simulink model "wturbines"  (R2024b)
settings: Solver=ode4  StartTime=0.0  StopTime=inf  FixedStep=0.01  RelTol=1e-3
values from neighbouring files (symbols this model uses):
  A_k = 2E6    (= 2000000)    [initialize_turbine_parameters.m]
  air_density = 1.225    [initialize_turbine_parameters.m]
  alpha_pitch_exp = 0    [initialize_turbine_parameters.m]
  B_k = 1E4    (= 10000)    [initialize_turbine_parameters.m]
  brake_torque = 28116.2    [initialize_turbine_parameters.m]
  C_k = 0    [initialize_turbine_parameters.m]
  Cp_mat = nan(numel(tsr_vec), numel(pitch_vec))    [initialize_turbine_parameters.m]
  Cp_opt = 0.482    [initialize_turbine_parameters.m]
  Ct_mat = nan(size(Cp_mat))    [initialize_turbine_parameters.m]
  ctrl_mode = 1    [initialize_turbine_parameters.m]
  cut_in_wind_speed = 3.0    (= 3)    [initialize_turbine_parameters.m]
  cut_out_wind_speed = 25.0    (= 25)    [initialize_turbine_parameters.m]
  D_k = 0    [initialize_turbine_parameters.m]
  dr_mode = Simulink.Parameter(1)    [initialize_turbine_parameters.m]
  gearbox_ratio = 1    [initialize_turbine_parameters.m]
  generator_eff = 0.954    [initialize_turbine_parameters.m]
  inertia = 1.9E6    (= 1900000)    [initialize_turbine_parameters.m]
  K_i_gen = 1e2    (= 100)    [initialize_turbine_parameters.m]
  K_i_pitch = 0    [initialize_turbine_parameters.m]
  K_i_pitch_gs = 0    [initialize_turbine_parameters.m]
  K_omega_sq = 1/2 * (tsr_opt)^-3 * air_density * pi * (rotor_diameter / 2)^5 * Cp_opt / gearbox_ratio^3    (= 69831977.2177)    [initialize_turbine_parameters.m]
  K_p_gen = 1e2    (= 100)    [initialize_turbine_parameters.m]
  K_p_pitch = 1    [initialize_turbine_parameters.m]
  K_p_pitch_gs = 0.1    [initialize_turbine_parameters.m]
  max_gen_torque = 1.15 * rated_gen_torque    (= 35686440.711)    [initialize_turbine_parameters.m]
  MIN_ROT_SPEED = 1e-3    (= 0.001)    [initialize_turbine_parameters.m]
  Nt = 9    [init.m]
  pitch_all = T{:, col_pitch}    [initialize_turbine_parameters.m]
  pitch_rate_deg = 5    [initialize_turbine_parameters.m]
  pitch_vec = sort(pitch_vec(:))    [initialize_turbine_parameters.m]
  rated_power = 22E6    (= 22000000)    [initialize_turbine_parameters.m]
  rated_rotor_speed = 6.77    [initialize_turbine_parameters.m]
  rated_rotor_speed_rads = rated_rotor_speed * (2 * pi) / 60    (= 0.70895274216)    [initialize_turbine_parameters.m]
  rated_wind_speed = 11.0    (= 11)    [initialize_turbine_parameters.m]
  ROT_EMG_MAX_TOL = 1.15    [initialize_turbine_parameters.m]
  ROT_SPEED_MIN_TRANS = min_rotor_speed_rads    (= 0.19)    [initialize_turbine_parameters.m]
  ROT_SPEED_SP_DIFF = 0.1    [initialize_turbine_parameters.m]
  rotor_radius = rotor_diameter / 2    (= 142)    [initialize_turbine_parameters.m]
  rotor_speed_all = [0, rated_rotor_speed]    [initialize_turbine_parameters.m]
  rotor_speed_init = rotor_speed_init * (2 * pi) / 60    (= 1.25663706144)    [initialize_turbine_parameters.m]
  rotor_speed_ref_mode = 1    [initialize_turbine_parameters.m]
  tsr_opt = 9.153    [initialize_turbine_parameters.m]
  tsr_vec = sort(tsr_vec(:))    [initialize_turbine_parameters.m]
  u_all = T{:, col_u}    [initialize_turbine_parameters.m]
  u_rotor_speed_all = [cut_in_wind_speed, rated_wind_speed]    [initialize_turbine_parameters.m]
  yawing_rate = 5    [initialize_turbine_parameters.m]
undefined symbols (not defined in the file or in its folder): op_mode, turbineDataBytes
libraries: simulink x24, simulink_extras x14, slpidlib x8, slrealtimeiplib x4, svdutilitieslib x2, slctrl_autotuning x2, etargetslib x2, dspstat3 x1
(part 2 of 3)

== system wturbines/For Each Subsystem/Turbine Dynamics + Controller1/Control logic/Power controller ==
  ws(t) : Inport
  ω(t) : Inport  Port=2
  P_set(t) : Inport  Port=3
  ω_g(t) : Inport  Port=4
  ctrl_mode : Inport  Port=5
  Demux : Demux  Outputs=2
  "Gain-scheduled H∞ control " : Subsystem
  Kω2 controller : Subsystem
  Lio downregulation : Subsystem
  Multiport Switch : MultiPortSwitch  Inputs=4  DataPortForDefault=Additional data port  SaturateOnIntegerOverflow=off  InputSameDT=off
  Mux{,1..3} (4 alike) : Mux  Inputs=2
  ROSCO : Subsystem
  T_g(t) : Outport
  β(t) : Outport  Port=2
  tag scope: ctrl_mode=global
  wires:
  Kω2 controller/1(T_g(t)) -> Mux/1
  Kω2 controller/2(β(t)) -> Mux/2
  ω(t)/1 -> Lio downregulation/1(ω(t)), "Gain-scheduled H∞ control "/1(ω_r(t))
  ws(t)/1 -> Kω2 controller/2(ws(t)), Lio downregulation/2(ws(t)), "Gain-scheduled H∞ control "/2(ws(t))
  P_set(t)/1 -> Lio downregulation/3(P_set(t))
  ctrl_mode/1 -> Multiport Switch/1, [ctrl_mode]
  Multiport Switch/1 -> Demux/1
  Demux/1 -> T_g(t)/1  "T_g(t)"
  Demux/2 -> β(t)/1  "β(t)"
  Lio downregulation/1(T_g(t)) -> Mux1/1
  Lio downregulation/2(β(t)) -> Mux1/2
  Mux/1 -> Multiport Switch/2
  Mux1/1 -> Multiport Switch/3
  ROSCO/2(β(t)) -> Mux2/2
  ROSCO/1(T_g(t)) -> Mux2/1
  "Gain-scheduled H∞ control "/1(T_g(t)) -> Mux3/1
  "Gain-scheduled H∞ control "/2(β(t)) -> Mux3/2
  Mux2/1 -> Multiport Switch/4
  Mux3/1 -> Multiport Switch/5
  ω_g(t)/1 -> Kω2 controller/1(ω(t))

== system wturbines/For Each Subsystem/Turbine Dynamics + Controller1/Turbine Dynamics/   ==
  rad : Inport
  Radians to Degrees : simulink_extras/Transformations/Radians to Degrees
  deg : Outport
  wires:
  rad/1 -> Radians to Degrees/1
  Radians to Degrees/1 -> deg/1

== system wturbines/For Each Subsystem/Turbine Dynamics + Controller1/Turbine Dynamics/      ==
  deg : Inport
  Degrees to Radians : simulink_extras/Transformations/Degrees to Radians
  rad : Outport
  wires:
  deg/1 -> Degrees to Radians/1
  Degrees to Radians/1 -> rad/1

== system wturbines/For Each Subsystem/Turbine Dynamics + Controller1/Turbine Dynamics/Collective Pitch Dynamics ==
  PtchSpt : Inport
  Rate Limiter : RateLimiter  RisingSlewLimit=pitch_rate_deg * (2 * pi / 360)  FallingSlewLimit=-pitch_rate_deg * (2 * pi / 360)  SampleTimeMode=inherited
  PitchAngle : Outport
  wires:
  PtchSpt/1 -> Rate Limiter/1
  Rate Limiter/1 -> PitchAngle/1

== system wturbines/For Each Subsystem/Turbine Dynamics + Controller1/Turbine Dynamics/Cp(λ, β) ==
  tsr : Inport
  pitch : Inport  Port=2
  Compare To Constant2 : simulink/Logic and Bit Operations/Compare To Constant  relop=<  const=min(pitch_vec)  OutDataTypeStr=boolean
  Compare To Constant3 : simulink/Logic and Bit Operations/Compare To Constant  relop=>  const=max(pitch_vec)  OutDataTypeStr=boolean
  Constant : Constant  Value=0
  "Cp(λ, β) " : Lookup_n-D  BreakpointsForDimension1=tsr_vec  BreakpointsForDimension2=pitch_vec  Table=Cp_mat  ExtrapMethod=Clip  DiagnosticForOutOfRangeInput=Error  InternalRulePriority=Speed  RndMeth=Simplest
      settings: InputPortMap=u0,u1
  OR1 : Logic  Operator=OR  IconShape=distinctive  AllPortsSameDT=off  OutDataTypeStr=boolean
  Saturation : Saturate  UpperLimit=1  LowerLimit=0
  Switch : Switch  Criteria=u2 ~= 0  SaturateOnIntegerOverflow=off  InputSameDT=off
  Cp : Outport
  wires:
  tsr/1 -> "Cp(λ, β) "/1
  pitch/1 -> "Cp(λ, β) "/2, Compare To Constant2/1, Compare To Constant3/1
  "Cp(λ, β) "/1 -> Switch/3  "Cp(t)"
  Compare To Constant2/1 -> OR1/1
  Compare To Constant3/1 -> OR1/2
  OR1/1 -> Switch/2
  Switch/1 -> Saturation/1
  Constant/1 -> Switch/1
  Saturation/1 -> Cp/1

== system wturbines/For Each Subsystem/Turbine Dynamics + Controller1/Turbine Dynamics/Orientation Dynamics ==
  OrientationSpt : Inport
  IC : InitialCondition  Value=270
  Rate Limiter : RateLimiter  RisingSlewLimit=yawing_rate  FallingSlewLimit=-yawing_rate  SampleTimeMode=inherited
  orientation : Outport
  wires:
  OrientationSpt/1 -> Rate Limiter/1  "psi_spt"
  Rate Limiter/1 -> IC/1
  IC/1 -> orientation/1

== system wturbines/For Each Subsystem/Turbine Dynamics + Controller1/Turbine Dynamics/P(t) ==
  ω(t) : Inport
  T_g(t) : Inport  Port=2
  Multiply : Gain  Gain=generator_eff
  Product : Product
  P(t) : Outport
  wires:
  ω(t)/1 -> Product/1
  T_g(t)/1 -> Product/2
  Multiply/1 -> P(t)/1
  Product/1 -> Multiply/1

== system wturbines/For Each Subsystem/Turbine Dynamics + Controller1/Turbine Dynamics/T_a(t) ==
  note: FIXME: This might have been the mistake,
      | which is fixed by this (missing) inverse
  ω(t) : Inport
  Cp(t) : Inport  Port=2
  ws(t) : Inport  Port=3
  "  " : Math  Operator=reciprocal  SignedPower=on
  Constant : Constant  Value=0.001
  Constant4 : Constant  Value=1/2
  Constant5 : Constant  Value=air_density
  Constant6 : Constant  Value=pi
  Constant7 : Constant  Value=rotor_radius
  Constant8 : Constant  Value=3
  Max : MinMax  Function=max  Inputs=2
  Power : Math  Operator=pow
  Product : Product  Inputs=7
  Saturation : Saturate  UpperLimit=inf  LowerLimit=0
  Square : Math  Operator=square
  T_a(t) : Outport
  wires:
  ω(t)/1 -> Max/1
  Product/1 -> Saturation/1  "T_a(t)"
  Square/1 -> Product/5
  Constant6/1 -> Product/6
  ws(t)/1 -> Power/1
  Constant5/1 -> Product/3
  Constant4/1 -> Product/2
  Power/1 -> Product/7
  Constant8/1 -> Power/2
  Constant7/1 -> Square/1
  Cp(t)/1 -> Product/4
  "  "/1 -> Product/1  "1/ω(t)"
  Constant/1 -> Max/2
  Max/1 -> "  "/1
  Saturation/1 -> T_a(t)/1

== system wturbines/For Each Subsystem/Turbine Dynamics + Controller1/Turbine Dynamics/λ(t) ==
  ω(t) : Inport
  ws(t) : Inport  Port=2
  Constant : Constant  Value=rotor_radius
  Divide : Product  Inputs=*/
  Product : Product
  λ(t) : Outport
  wires:
  ws(t)/1 -> Divide/2
  Product/1 -> Divide/1
  ω(t)/1 -> Product/1
  Divide/1 -> λ(t)/1  "λ(t)"
  Constant/1 -> Product/2

== system wturbines/For Each Subsystem/Turbine Dynamics + Controller/Power controller/Gain-scheduled H∞ control /  ==
  rpm : Inport
  Multiply : Gain  Gain=2 * pi
  Multiply1 : Gain  Gain=1 / 60
  rad/s : Outport
  wires:
  Multiply1/1 -> rad/s/1
  rpm/1 -> Multiply/1
  Multiply/1 -> Multiply1/1

== system wturbines/For Each Subsystem/Turbine Dynamics + Controller/Power controller/Gain-scheduled H∞ control /   ==
  rpm : Inport
  Multiply : Gain  Gain=2 * pi
  Multiply1 : Gain  Gain=1 / 60
  rad/s : Outport
  wires:
  Multiply1/1 -> rad/s/1
  rpm/1 -> Multiply/1
  Multiply/1 -> Multiply1/1

== system wturbines/For Each Subsystem/Turbine Dynamics + Controller/Power controller/Gain-scheduled H∞ control /Pitch controller ==
  e_ω,r(t) : Inport
  β(t) : Inport  Port=2
  Bus Creator : BusCreator  Inputs=2
  Gain : Gain  Gain=K_p_pitch_gs
  Gain scheduler : slctrl_autotuning/PID Gain Scheduler  ControllerType=PI  BPsInGainArray=off  GainArrayBreakpoints=[0 30]  UseExternalBreakpoints=off  GainSourceMethod=Input to block  StoreGainsPParamName=PGain  StoreGainsIParamName=IGain  StoreGainsDParamName=DGain  StoreGainsNParamName=NGain  BlockDataType=Double  PGainLookUpMeth=Interpolation-Use End Values  IGainLookUpMeth=Interpolation-Use End Values  DGainLookUpMeth=Interpolation-Use End Values  NGainLookUpMeth=Interpolation-Use End Values  DoSatur=off  BreakpointSourceLookupVariant=InternalBPs  GainSourceVariant=External  BreakpointSourceVariant=InternalBPs  PGainVariant=Enabled  IGainVariant=Enabled  DGainVariant=Disabled  NGainVariant=Disabled
      settings: LibrarySourceBlock=slctrlblks/Autotuning/PID Gain Scheduler
  Gain1 : Gain  Gain=K_i_pitch_gs
  Gains : Constant  Value=[1 3]
  PI Controller : slpidlib/PID Controller  Controller=PI  Form=Parallel  TimeDomain=Continuous-time  UseExternalTs=off  SampleTime=-1  IntegratorMethod=Forward Euler  FilterMethod=Forward Euler  ControllerParametersSource=external  P=1  I=1  UseKiTs=off  D=0  UseExternalDerivativeSource=off  N=100  UseFilter=on  TunerSelectOption=Transfer Function Based (PID Tuner App)  InitialConditionSource=internal  InitialConditionForIntegrator=0  InitialConditionForFilter=0  DifferentiatorICPrevScaledInput=0  ExternalReset=none  TrackingMode=off  Kt=1  LimitOutput=off  SatLimitsSource=internal  UpperSaturationLimit=inf  LowerSaturationLimit=-inf  LinearizeAsGain=on  AntiWindupMode=none  Kb=1  LimitIntegrator=off  UpperIntegratorSaturationLimit=inf  LowerIntegratorSaturationLimit=-inf  POutMin=[]  POutMax=[]  IOutMin=[]  IOutMax=[]  DOutMin=[]  DOutMax=[]  NOutMin=[]  NOutMax=[]  SumOutMin=[]  SumOutMax=[]  SaturationOutMin=[]  SaturationOutMax=[]  PParamMin=[]  PParamMax=[]  IParamMin=[]  IParamMax=[]  DParamMin=[]  DParamMax=[]  NParamMin=[]  NParamMax=[]  KbParamMin=[]  KbParamMax=[]  KtParamMin=[]  KtParamMax=[]  KbOutMin=[]  KbOutMax=[]  KtOutMin=[]  KtOutMax=[]  IntegratorOutMin=[]  IntegratorOutMax=[]  FilterOutMin=[]  FilterOutMax=[]  SumI1OutMin=[]  SumI1OutMax=[]  SumI2OutMin=[]  SumI2OutMax=[]  SumI3OutMin=[]  SumI3OutMax=[]  SumI4OutMin=[]  SumI4OutMax=[]  SumDOutMin=[]  SumDOutMax=[]  DifferentiatorOutMin=[]  DifferentiatorOutMax=[]  FilterDiffOutCoefMin=[]  FilterDiffOutCoefMax=[]  ReciprocalOutMin=[]  ReciprocalOutMax=[]  SumDenOutMin=[]  SumDenOutMax=[]  SumNumOutMin=[]  SumNumOutMax=[]  DivideOutMin=[]  DivideOutMax=[]  UdiffTsProdOutMin=[]  UdiffTsProdOutMax=[]  NTsProdOutMin=[]  NTsProdOutMax=[]  UintegralTsProdOutMin=[]  UintegralTsProdOutMax=[]  UngainTsProdOutMin=[]  UngainTsProdOutMax=[]  ClampingZeroOutDataTypeStr=Inherit: Inherit via back propagation  ClampingZeroOutMin=[]  ClampingZeroOutMax=[]  FilterDenConstantOutDataTypeStr=Inherit: Inherit via back propagation  FilterDenConstantOutMin=[]  FilterDenConstantOutMax=[]  PCopyOutDataTypeStr=Inherit: Inherit via back propagation  PCopyOutMin=[]  PCopyOutMax=[]  NCopyOutDataTypeStr=Inherit: Inherit via back propagation  NCopyOutMin=[]  NCopyOutMax=[]  IntegratorContinuousStateAttributes=''  IntegratorStateMustResolveToSignalObject=off  IntegratorRTWStateStorageClass=Auto  FilterContinuousStateAttributes=''  FilterStateMustResolveToSignalObject=off  FilterRTWStateStorageClass=Auto  ParallelPVariant=ExternalParameters  IdealPVariant=Disabled  IVariant=ExternalParameters  DVariant=Disabled  IntegratorVariant=Continuous  SatVariant=Disabled  AWVariant=Passthrough  PCopyVariant=Disabled  TRVariant=Disabled  FdbkBlocksVariant=Forward  IdealPFdbkVariant=Disabled  SatFdbkVariant=Disabled  DerivativeFilterVariant=Disabled  NVariant=Disabled  NCopyVariant=Disabled_SignalSpec  FilterICVariant=Disabled  IntegratorICVariant=InternalICs  ExternalResetVariant=Disabled  TRSumVariant=Passthrough  SumFdbkVariant=Disabled  SumVariant=Sum_PI  TsampFilterVariant=InternalTs  TsampNgainVariant=Passthrough  TsampIntegralVariant=Disabled_SignalSpec  ExternalSaturationOutDataTypeStr=Inherit: Same as second input  DerivativeSourceVariant=Disabled  PreIntVariant=InternalPreInt
  Signal Copy : SignalConversion  OverrideOpt=off
  rad2deg : Subsystem
  β_ref(t) : Outport
  wires:
  Signal Copy/1 -> Bus Creator/2  "I"
  β(t)/1 -> rad2deg/1(rad)
  rad2deg/1(deg) -> Gain scheduler/1  "β(t)"
  Gains/1 -> Bus Creator/1, Signal Copy/1  "P"
  Bus Creator/1 -> Gain scheduler/2
  Gain1/1 -> PI Controller/3
  Gain/1 -> PI Controller/2
  Gain scheduler/2 -> Gain1/1
  Gain scheduler/1 -> Gain/1
  PI Controller/1 -> β_ref(t)/1
  e_ω,r(t)/1 -> PI Controller/1

== system wturbines/For Each Subsystem/Turbine Dynamics + Controller/Power controller/Gain-scheduled H∞ control /Torque controller ==
  note: Temporary workaround
  e_ω,r(t) : Inport
  "H∞ controller " : StateSpace  A=A_k  B=B_k  C=C_k  D=D_k  InitialCondition=0
  PI controller : slpidlib/PID Controller  Controller=PI  Form=Parallel  TimeDomain=Continuous-time  UseExternalTs=off  SampleTime=-1  IntegratorMethod=Forward Euler  FilterMethod=Forward Euler  ControllerParametersSource=internal  P=A_k  I=B_k  UseKiTs=off  D=0  UseExternalDerivativeSource=off  N=100  UseFilter=on  TunerSelectOption=Transfer Function Based (PID Tuner App)  InitialConditionSource=internal  InitialConditionForIntegrator=0  InitialConditionForFilter=0  DifferentiatorICPrevScaledInput=0  ExternalReset=none  TrackingMode=off  Kt=1  LimitOutput=off  SatLimitsSource=internal  UpperSaturationLimit=inf  LowerSaturationLimit=-inf  LinearizeAsGain=on  AntiWindupMode=none  Kb=1  LimitIntegrator=off  UpperIntegratorSaturationLimit=inf  LowerIntegratorSaturationLimit=-inf  POutMin=[]  POutMax=[]  IOutMin=[]  IOutMax=[]  DOutMin=[]  DOutMax=[]  NOutMin=[]  NOutMax=[]  SumOutMin=[]  SumOutMax=[]  SaturationOutMin=[]  SaturationOutMax=[]  PParamMin=[]  PParamMax=[]  IParamMin=[]  IParamMax=[]  DParamMin=[]  DParamMax=[]  NParamMin=[]  NParamMax=[]  KbParamMin=[]  KbParamMax=[]  KtParamMin=[]  KtParamMax=[]  KbOutMin=[]  KbOutMax=[]  KtOutMin=[]  KtOutMax=[]  IntegratorOutMin=[]  IntegratorOutMax=[]  FilterOutMin=[]  FilterOutMax=[]  SumI1OutMin=[]  SumI1OutMax=[]  SumI2OutMin=[]  SumI2OutMax=[]  SumI3OutMin=[]  SumI3OutMax=[]  SumI4OutMin=[]  SumI4OutMax=[]  SumDOutMin=[]  SumDOutMax=[]  DifferentiatorOutMin=[]  DifferentiatorOutMax=[]  FilterDiffOutCoefMin=[]  FilterDiffOutCoefMax=[]  ReciprocalOutMin=[]  ReciprocalOutMax=[]  SumDenOutMin=[]  SumDenOutMax=[]  SumNumOutMin=[]  SumNumOutMax=[]  DivideOutMin=[]  DivideOutMax=[]  UdiffTsProdOutMin=[]  UdiffTsProdOutMax=[]  NTsProdOutMin=[]  NTsProdOutMax=[]  UintegralTsProdOutMin=[]  UintegralTsProdOutMax=[]  UngainTsProdOutMin=[]  UngainTsProdOutMax=[]  ClampingZeroOutDataTypeStr=Inherit: Inherit via back propagation  ClampingZeroOutMin=[]  ClampingZeroOutMax=[]  FilterDenConstantOutDataTypeStr=Inherit: Inherit via back propagation  FilterDenConstantOutMin=[]  FilterDenConstantOutMax=[]  PCopyOutDataTypeStr=Inherit: Inherit via back propagation  PCopyOutMin=[]  PCopyOutMax=[]  NCopyOutDataTypeStr=Inherit: Inherit via back propagation  NCopyOutMin=[]  NCopyOutMax=[]  IntegratorContinuousStateAttributes=''  IntegratorStateMustResolveToSignalObject=off  IntegratorRTWStateStorageClass=Auto  FilterContinuousStateAttributes=''  FilterStateMustResolveToSignalObject=off  FilterRTWStateStorageClass=Auto  ParallelPVariant=InternalParameters  IdealPVariant=Disabled  IVariant=InternalParameters  DVariant=Disabled  IntegratorVariant=Continuous  SatVariant=Disabled  AWVariant=Passthrough  PCopyVariant=Disabled  TRVariant=Disabled  FdbkBlocksVariant=Forward  IdealPFdbkVariant=Disabled  SatFdbkVariant=Disabled  DerivativeFilterVariant=Disabled  NVariant=Disabled  NCopyVariant=Disabled_SignalSpec  FilterICVariant=Disabled  IntegratorICVariant=InternalICs  ExternalResetVariant=Disabled  TRSumVariant=Passthrough  SumFdbkVariant=Disabled  SumVariant=Sum_PI  TsampFilterVariant=InternalTs  TsampNgainVariant=Passthrough  TsampIntegralVariant=Disabled_SignalSpec  ExternalSaturationOutDataTypeStr=Inherit: Same as second input  DerivativeSourceVariant=Disabled  PreIntVariant=InternalPreInt
  T_g(t) : Outport
  wires:
  "H∞ controller "/1 -> ?
  PI controller/1 -> T_g(t)/1
  e_ω,r(t)/1 -> PI controller/1

== system wturbines/For Each Subsystem/Turbine Dynamics + Controller/Power controller/Kω2 controller/Pitch controller ==
  ws(t) : Inport
  ω(t) : Inport  Port=2
  "  " : Subsystem
  Constant : Constant  Value=rated_rotor_speed
  Constant1 : Constant  Value=alpha_pitch_exp
  Constant2 : Constant  Value=0
  Exp : Math
  IsNaN1 : RelationalOperator  Operator=isNaN  OutDataTypeStr=boolean  RndMeth=Simplest  InputSameDT=off
  NOT : Logic  Operator=NOT  IconShape=distinctive  AllPortsSameDT=off  OutDataTypeStr=boolean
  Product : Product
  Product1 : Product
  Sum : Sum  Inputs=|+-
  Switch : Switch  Criteria=u2 ~= 0  SaturateOnIntegerOverflow=off  InputSameDT=off
  rad2deg : Subsystem
  β(ws) : Lookup_n-D  NumberOfTableDimensions=1  BreakpointsForDimension1=u_all  Table=pitch_all  InternalRulePriority=Speed  RndMeth=Simplest
  β(t) : Outport
  wires:
  Switch/1 -> β(t)/1
  NOT/1 -> Switch/2  "is_not_nan"
  Product/1 -> IsNaN1/1, Switch/1
  Constant2/1 -> Switch/3
  IsNaN1/1 -> NOT/1
  "  "/1(rad/s) -> Sum/2  "ω_rated"
  rad2deg/1(rad) -> Product/1  "β(t)"
  Constant1/1 -> Product1/2
  Product1/1 -> Exp/1
  Sum/1 -> Product1/1
  Exp/1 -> Product/2
  Constant/1 -> "  "/1(rpm)
  ω(t)/1 -> Sum/1
  ws(t)/1 -> β(ws)/1
  β(ws)/1 -> rad2deg/1(deg)

== system wturbines/For Each Subsystem/Turbine Dynamics + Controller/Power controller/Kω2 controller/Torque controller ==
  ω(t) : Inport
  Constant : Constant  Value=K_omega_sq
  Product : Product
  Square : Math  Operator=square
  T_g(t) : Outport
  wires:
  Constant/1 -> Product/2
  Product/1 -> T_g(t)/1
  Square/1 -> Product/1
  ω(t)/1 -> Square/1

== system wturbines/For Each Subsystem/Turbine Dynamics + Controller/Power controller/Lio downregulation/   ==
  rpm : Inport
  Multiply : Gain  Gain=2 * pi
  Multiply1 : Gain  Gain=1 / 60
  rad/s : Outport
  wires:
  Multiply1/1 -> rad/s/1
  rpm/1 -> Multiply/1
  Multiply/1 -> Multiply1/1

== system wturbines/For Each Subsystem/Turbine Dynamics + Controller/Power controller/Lio downregulation/Pitch controller ==
  ws(t) : Inport
  ws_dr(t) : Inport  Port=2
  e_ω(t) : Inport  Port=3
  Constant : Constant  Value=0
  Derating : Switch  Criteria=u2 > Threshold  SaturateOnIntegerOverflow=off  InputSameDT=off
  PI controller : slpidlib/PID Controller  Controller=PI  Form=Parallel  TimeDomain=Continuous-time  UseExternalTs=off  SampleTime=-1  IntegratorMethod=Forward Euler  FilterMethod=Forward Euler  ControllerParametersSource=internal  P=K_p_pitch  I=K_i_pitch  UseKiTs=off  D=0  UseExternalDerivativeSource=off  N=100  UseFilter=on  TunerSelectOption=Transfer Function Based (PID Tuner App)  InitialConditionSource=internal  InitialConditionForIntegrator=0  InitialConditionForFilter=0  DifferentiatorICPrevScaledInput=0  ExternalReset=none  TrackingMode=off  Kt=1  LimitOutput=off  SatLimitsSource=internal  UpperSaturationLimit=inf  LowerSaturationLimit=-inf  LinearizeAsGain=on  AntiWindupMode=none  Kb=1  LimitIntegrator=off  UpperIntegratorSaturationLimit=inf  LowerIntegratorSaturationLimit=-inf  POutMin=[]  POutMax=[]  IOutMin=[]  IOutMax=[]  DOutMin=[]  DOutMax=[]  NOutMin=[]  NOutMax=[]  SumOutMin=[]  SumOutMax=[]  SaturationOutMin=[]  SaturationOutMax=[]  PParamMin=[]  PParamMax=[]  IParamMin=[]  IParamMax=[]  DParamMin=[]  DParamMax=[]  NParamMin=[]  NParamMax=[]  KbParamMin=[]  KbParamMax=[]  KtParamMin=[]  KtParamMax=[]  KbOutMin=[]  KbOutMax=[]  KtOutMin=[]  KtOutMax=[]  IntegratorOutMin=[]  IntegratorOutMax=[]  FilterOutMin=[]  FilterOutMax=[]  SumI1OutMin=[]  SumI1OutMax=[]  SumI2OutMin=[]  SumI2OutMax=[]  SumI3OutMin=[]  SumI3OutMax=[]  SumI4OutMin=[]  SumI4OutMax=[]  SumDOutMin=[]  SumDOutMax=[]  DifferentiatorOutMin=[]  DifferentiatorOutMax=[]  FilterDiffOutCoefMin=[]  FilterDiffOutCoefMax=[]  ReciprocalOutMin=[]  ReciprocalOutMax=[]  SumDenOutMin=[]  SumDenOutMax=[]  SumNumOutMin=[]  SumNumOutMax=[]  DivideOutMin=[]  DivideOutMax=[]  UdiffTsProdOutMin=[]  UdiffTsProdOutMax=[]  NTsProdOutMin=[]  NTsProdOutMax=[]  UintegralTsProdOutMin=[]  UintegralTsProdOutMax=[]  UngainTsProdOutMin=[]  UngainTsProdOutMax=[]  ClampingZeroOutDataTypeStr=Inherit: Inherit via back propagation  ClampingZeroOutMin=[]  ClampingZeroOutMax=[]  FilterDenConstantOutDataTypeStr=Inherit: Inherit via back propagation  FilterDenConstantOutMin=[]  FilterDenConstantOutMax=[]  PCopyOutDataTypeStr=Inherit: Inherit via back propagation  PCopyOutMin=[]  PCopyOutMax=[]  NCopyOutDataTypeStr=Inherit: Inherit via back propagation  NCopyOutMin=[]  NCopyOutMax=[]  IntegratorContinuousStateAttributes=''  IntegratorStateMustResolveToSignalObject=off  IntegratorRTWStateStorageClass=Auto  FilterContinuousStateAttributes=''  FilterStateMustResolveToSignalObject=off  FilterRTWStateStorageClass=Auto  ParallelPVariant=InternalParameters  IdealPVariant=Disabled  IVariant=InternalParameters  DVariant=Disabled  IntegratorVariant=Continuous  SatVariant=Disabled  AWVariant=Passthrough  PCopyVariant=Disabled  TRVariant=Disabled  FdbkBlocksVariant=Forward  IdealPFdbkVariant=Disabled  SatFdbkVariant=Disabled  DerivativeFilterVariant=Disabled  NVariant=Disabled  NCopyVariant=Disabled_SignalSpec  FilterICVariant=Disabled  IntegratorICVariant=InternalICs  ExternalResetVariant=Disabled  TRSumVariant=Passthrough  SumFdbkVariant=Disabled  SumVariant=Sum_PI  TsampFilterVariant=InternalTs  TsampNgainVariant=Passthrough  TsampIntegralVariant=Disabled_SignalSpec  ExternalSaturationOutDataTypeStr=Inherit: Same as second input  DerivativeSourceVariant=Disabled  PreIntVariant=InternalPreInt
  Sum : Sum  Inputs=-+|
  β(t) : Outport
  wires:
  PI controller/1 -> Derating/3
  Constant/1 -> Derating/1
  e_ω(t)/1 -> PI controller/1
  Sum/1 -> Derating/2  "(ws_dr - ws)(t)"
  ws(t)/1 -> Sum/1
  ws_dr(t)/1 -> Sum/2
  Derating/1 -> β(t)/1

== system wturbines/For Each Subsystem/Turbine Dynamics + Controller/Power controller/Lio downregulation/Torque controller ==
  ω_set(t) : Inport
  ws(t) : Inport  Port=2
  ws_dr(t) : Inport  Port=3
  e_ω(t) : Inport  Port=4
  P_set(t) : Inport  Port=5
  Derating : Switch  Criteria=u2 > Threshold  SaturateOnIntegerOverflow=off  InputSameDT=off
  Divide : Product  Inputs=*/
  PI controller : slpidlib/PID Controller  Controller=PI  Form=Parallel  TimeDomain=Continuous-time  UseExternalTs=off  SampleTime=-1  IntegratorMethod=Forward Euler  FilterMethod=Forward Euler  ControllerParametersSource=internal  P=K_p_gen  I=K_i_gen  UseKiTs=off  D=0  UseExternalDerivativeSource=off  N=100  UseFilter=on  TunerSelectOption=Transfer Function Based (PID Tuner App)  InitialConditionSource=internal  InitialConditionForIntegrator=0  InitialConditionForFilter=0  DifferentiatorICPrevScaledInput=0  ExternalReset=none  TrackingMode=off  Kt=1  LimitOutput=off  SatLimitsSource=internal  UpperSaturationLimit=inf  LowerSaturationLimit=-inf  LinearizeAsGain=on  AntiWindupMode=none  Kb=1  LimitIntegrator=off  UpperIntegratorSaturationLimit=inf  LowerIntegratorSaturationLimit=-inf  POutMin=[]  POutMax=[]  IOutMin=[]  IOutMax=[]  DOutMin=[]  DOutMax=[]  NOutMin=[]  NOutMax=[]  SumOutMin=[]  SumOutMax=[]  SaturationOutMin=[]  SaturationOutMax=[]  PParamMin=[]  PParamMax=[]  IParamMin=[]  IParamMax=[]  DParamMin=[]  DParamMax=[]  NParamMin=[]  NParamMax=[]  KbParamMin=[]  KbParamMax=[]  KtParamMin=[]  KtParamMax=[]  KbOutMin=[]  KbOutMax=[]  KtOutMin=[]  KtOutMax=[]  IntegratorOutMin=[]  IntegratorOutMax=[]  FilterOutMin=[]  FilterOutMax=[]  SumI1OutMin=[]  SumI1OutMax=[]  SumI2OutMin=[]  SumI2OutMax=[]  SumI3OutMin=[]  SumI3OutMax=[]  SumI4OutMin=[]  SumI4OutMax=[]  SumDOutMin=[]  SumDOutMax=[]  DifferentiatorOutMin=[]  DifferentiatorOutMax=[]  FilterDiffOutCoefMin=[]  FilterDiffOutCoefMax=[]  ReciprocalOutMin=[]  ReciprocalOutMax=[]  SumDenOutMin=[]  SumDenOutMax=[]  SumNumOutMin=[]  SumNumOutMax=[]  DivideOutMin=[]  DivideOutMax=[]  UdiffTsProdOutMin=[]  UdiffTsProdOutMax=[]  NTsProdOutMin=[]  NTsProdOutMax=[]  UintegralTsProdOutMin=[]  UintegralTsProdOutMax=[]  UngainTsProdOutMin=[]  UngainTsProdOutMax=[]  ClampingZeroOutDataTypeStr=Inherit: Inherit via back propagation  ClampingZeroOutMin=[]  ClampingZeroOutMax=[]  FilterDenConstantOutDataTypeStr=Inherit: Inherit via back propagation  FilterDenConstantOutMin=[]  FilterDenConstantOutMax=[]  PCopyOutDataTypeStr=Inherit: Inherit via back propagation  PCopyOutMin=[]  PCopyOutMax=[]  NCopyOutDataTypeStr=Inherit: Inherit via back propagation  NCopyOutMin=[]  NCopyOutMax=[]  IntegratorContinuousStateAttributes=''  IntegratorStateMustResolveToSignalObject=off  IntegratorRTWStateStorageClass=Auto  FilterContinuousStateAttributes=''  FilterStateMustResolveToSignalObject=off  FilterRTWStateStorageClass=Auto  ParallelPVariant=InternalParameters  IdealPVariant=Disabled  IVariant=InternalParameters  DVariant=Disabled  IntegratorVariant=Continuous  SatVariant=Disabled  AWVariant=Passthrough  PCopyVariant=Disabled  TRVariant=Disabled  FdbkBlocksVariant=Forward  IdealPFdbkVariant=Disabled  SatFdbkVariant=Disabled  DerivativeFilterVariant=Disabled  NVariant=Disabled  NCopyVariant=Disabled_SignalSpec  FilterICVariant=Disabled  IntegratorICVariant=InternalICs  ExternalResetVariant=Disabled  TRSumVariant=Passthrough  SumFdbkVariant=Disabled  SumVariant=Sum_PI  TsampFilterVariant=InternalTs  TsampNgainVariant=Passthrough  TsampIntegralVariant=Disabled_SignalSpec  ExternalSaturationOutDataTypeStr=Inherit: Same as second input  DerivativeSourceVariant=Disabled  PreIntVariant=InternalPreInt
  Sum : Sum  Inputs=-+|
  T_g(t) : Outport
  wires:
  Divide/1 -> Derating/3
  PI controller/1 -> Derating/1
  ω_set(t)/1 -> Divide/2
  P_set(t)/1 -> Divide/1
  Derating/1 -> T_g(t)/1
  ws(t)/1 -> Sum/1
  e_ω(t)/1 -> PI controller/1
  ws_dr(t)/1 -> Sum/2
  Sum/1 -> Derating/2  "(ws_dr - ws)(t)"

== system wturbines/For Each Subsystem/Turbine Dynamics + Controller/Power controller/Lio downregulation/rads2rpm ==
  rad/s : Inport
  Multiply : Gain  Gain=1 / (2 * pi)
  Multiply1 : Gain  Gain=60
  rpm : Outport
  wires:
  Multiply1/1 -> rpm/1
  rad/s/1 -> Multiply/1
  Multiply/1 -> Multiply1/1

== system wturbines/For Each Subsystem/Turbine Dynamics + Controller/Power controller/ROSCO/Pitch controller ==
  ω_g(t) : Inport
  Δω_g(t) : Inport  Port=2
  β_min(t) : Inport  Port=3
  Constant : Constant  Value=rated_rotor_speed
  Gain : Gain  Gain=gearbox_ratio
  β(t) : Outport
  wires:
  Gain/1 -> ?  "ω_g,rated"
  Constant/1 -> Gain/1

== system wturbines/For Each Subsystem/Turbine Dynamics + Controller/Power controller/ROSCO/Torque controller ==
  ω_g(t) : Inport
  ws(t) : Inport  Port=2
  Δω_g(t) : Inport  Port=3
  β(t) : Inport  Port=4
  T_g(t) : Outport

== system wturbines/For Each Subsystem/Turbine Dynamics + Controller1/Control logic/Power controller/Gain-scheduled H∞ control  ==
  note: To prevent algebraic loop
  note: Actuator dynamics
  note: 3 | Constant-TSR
  note: 2 | Max-ω
  note: * | Shutdown
  note: 1 | Steady-state lookup
  ω_r(t) : Inport
  ws(t) : Inport  Port=2
  " " : Subsystem
  "  " : Subsystem
  Constant11 : Constant  Value=rotor_radius
  Constant12 : Constant  Value=tsr_opt
  Constant13 : Constant  Value=0
  Delay : Delay  DelayLength=1
  Divide4 : Product  Inputs=**/
  Mode : Constant  Value=rotor_speed_ref_mode
  Multiport Switch : MultiPortSwitch  DataPortForDefault=Additional data port  DiagnosticForDefault=None  SaturateOnIntegerOverflow=off  InputSameDT=off
  Pitch controller : Subsystem
  Sum : Sum  Inputs=|+-
  Torque controller : Subsystem
  ω_set : Constant  Value=rated_rotor_speed
  ω_ss(u) : Lookup_n-D  NumberOfTableDimensions=1  BreakpointsForDimension1=u_rotor_speed_all  Table=rotor_speed_all  InternalRulePriority=Speed  RndMeth=Simplest
  T_g(t) : Outport
  β(t) : Outport  Port=2
  wires:
  Torque controller/1(T_g(t)) -> T_g(t)/1
  Pitch controller/1(β_ref(t)) -> Delay/1, β(t)/1
  Delay/1 -> Pitch controller/2(β(t))
  Sum/1 -> Pitch controller/1(e_ω,r(t)), Torque controller/1(e_ω,r(t))  "e_ω,r(t)"
  Constant12/1 -> Divide4/1
  Mode/1 -> Multiport Switch/1
  Constant11/1 -> Divide4/3
  Divide4/1 -> Multiport Switch/4  "ω_r,ref(t)"
  Constant13/1 -> Multiport Switch/5
  ω_set/1 -> "  "/1(rpm)  "ω_rated"
  Multiport Switch/1 -> Sum/2  "ω_r,ref(t)"
  ω_r(t)/1 -> Sum/1
  ws(t)/1 -> ω_ss(u)/1, Divide4/2  "ws(t)"
  ω_ss(u)/1 -> " "/1(rpm)  "ω_ss(t)"
  " "/1(rad/s) -> Multiport Switch/2  "ω_ss(t)"
  "  "/1(rad/s) -> Multiport Switch/3  "ω_rated"

== system wturbines/For Each Subsystem/Turbine Dynamics + Controller1/Control logic/Power controller/Kω2 controller ==
  ω(t) : Inport
  ws(t) : Inport  Port=2
  Pitch controller : Subsystem
  Torque controller : Subsystem
  T_g(t) : Outport
  β(t) : Outport  Port=2
  wires:
  Torque controller/1(T_g(t)) -> [KomegaGen], T_g(t)/1
  Pitch controller/1(β(t)) -> β(t)/1
  ω(t)/1 -> Pitch controller/2(ω(t)), Torque controller/1(ω(t))
  ws(t)/1 -> Torque controller/2(ws), Pitch controller/1(ws(t))

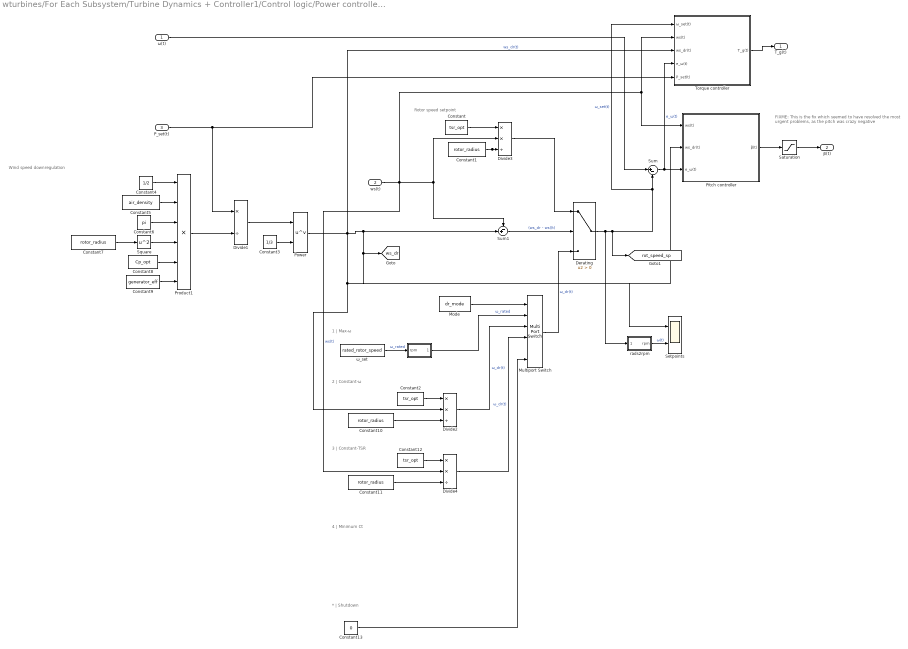
== system wturbines/For Each Subsystem/Turbine Dynamics + Controller1/Control logic/Power controller/Lio downregulation ==
  note: 1 | Max-ω
  note: Wind speed downregulation
  note: Rotor speed setpoint
  note: 2 | Constant-ω
  note: 3 | Constant-TSR
  note: 4 | Minimum Ct
  note: * | Shutdown
  note: FIXME: This is the fix which seemed to have resolved
      | the most urgent problems, as the pitch was crazy negative
  ω(t) : Inport
  ws(t) : Inport  Port=2
  P_set(t) : Inport  Port=3
  "  " : Subsystem
  Constant : Constant  Value=tsr_opt
  Constant{1,7,10..11} (4 alike) : Constant  Value=rotor_radius
  Constant12 : Constant  Value=tsr_opt
  Constant13 : Constant  Value=0
  Constant2 : Constant  Value=tsr_opt
  Constant3 : Constant  Value=1/3
  Constant4 : Constant  Value=1/2
  Constant5 : Constant  Value=air_density
  Constant6 : Constant  Value=pi
  Constant8 : Constant  Value=Cp_opt
  Constant9 : Constant  Value=generator_eff
  Derating : Switch  Criteria=u2 > Threshold  SaturateOnIntegerOverflow=off  InputSameDT=off
  Divide1 : Product  Inputs=*/
  Divide2 : Product  Inputs=**/
  Divide3 : Product  Inputs=**/
  Divide4 : Product  Inputs=**/
  Mode : Constant  Value=dr_mode
  Multiport Switch : MultiPortSwitch  Inputs=4  DataPortForDefault=Additional data port  DiagnosticForDefault=None  SaturateOnIntegerOverflow=off  InputSameDT=off
  Pitch controller : Subsystem
  Power : Math  Operator=pow
  Product1 : Product  Inputs=6
  Saturation : Saturate  UpperLimit=90 * (2 * pi / 360)  LowerLimit=-2 * (2 * pi / 360)
  Setpoints : Scope  NumInputPorts=2
  Square : Math  Operator=square
  Sum : Sum  Inputs=|+-
  Sum1 : Sum  Inputs=-+|
  Torque controller : Subsystem
  rads2rpm : Subsystem
  ω_set : Constant  Value=rated_rotor_speed
  T_g(t) : Outport
  β(t) : Outport  Port=2
  tag scope: rot_speed_sp=global, ws_dr=global
  wires:
  Torque controller/1(T_g(t)) -> T_g(t)/1
  Pitch controller/1(β(t)) -> Saturation/1
  Derating/1 -> rads2rpm/1(rad/s), Torque controller/1(ω_set(t)), Sum/2, [rot_speed_sp]  "ω_set(t)"
  Sum/1 -> Torque controller/4(e_ω(t)), Pitch controller/3(e_ω(t))  "e_ω(t)"
  Divide3/1 -> Derating/1
  Constant1/1 -> Divide3/3
  Constant/1 -> Divide3/1
  Sum1/1 -> Derating/2  "(ws_dr - ws)(t)"
  Power/1 -> Sum1/2, [ws_dr], Setpoints/1, Divide2/2, Pitch controller/2(ws_dr(t)), Torque controller/3(ws_dr(t))  "ws_dr(t)"
  ws(t)/1 -> Divide4/2, Pitch controller/1(ws(t)), Torque controller/2(ws(t)), Divide3/2, Sum1/1  "ws(t)"
  Constant3/1 -> Power/2
  P_set(t)/1 -> Torque controller/5(P_set(t)), Divide1/1
  Divide1/1 -> Power/1
  Product1/1 -> Divide1/2
  Constant4/1 -> Product1/1
  Constant5/1 -> Product1/2
  Constant6/1 -> Product1/3
  Constant7/1 -> Square/1
  Square/1 -> Product1/4
  Constant8/1 -> Product1/5
  Constant9/1 -> Product1/6
  ω(t)/1 -> Sum/1
  ω_set/1 -> "  "/1(rpm)  "ω_rated"
  Divide2/1 -> Multiport Switch/3  "ω_dr(t)"
  Constant2/1 -> Divide2/1
  Constant10/1 -> Divide2/3
  Multiport Switch/1 -> Derating/3  "ω_dr(t)"
  Mode/1 -> Multiport Switch/1
  Constant11/1 -> Divide4/3
  Constant12/1 -> Divide4/1
  Divide4/1 -> Multiport Switch/4  "ω_dr(t)"
  Constant13/1 -> Multiport Switch/6
  rads2rpm/1(rpm) -> Setpoints/2  "ω(t)"
  "  "/1(rad/s) -> Multiport Switch/2  "ω_rated"
  Saturation/1 -> β(t)/1

== system wturbines/For Each Subsystem/Turbine Dynamics + Controller1/Control logic/Power controller/ROSCO ==
  note: Setpoint smoother
  note: Pitch saturation
  ω_r(t) : Inport
  ws(t) : Inport  Port=2
  ω_g(t) : Inport  Port=3
  Pitch controller : Subsystem
  Torque controller : Subsystem
  T_g(t) : Outport
  β(t) : Outport  Port=2
  wires:
  Torque controller/1(T_g(t)) -> T_g(t)/1
  Pitch controller/1(β(t)) -> Torque controller/4(β(t)), β(t)/1
  ? -> Torque controller/3(Δω_g(t)), Pitch controller/2(Δω_g(t))  "Δω_g(t)"

== system wturbines/For Each Subsystem/Turbine Dynamics + Controller/Power controller/Gain-scheduled H∞ control /Pitch controller/rad2deg ==
  rad : Inport
  Radians to Degrees : simulink_extras/Transformations/Radians to Degrees
  deg : Outport
  wires:
  Radians to Degrees/1 -> deg/1
  rad/1 -> Radians to Degrees/1

== system wturbines/For Each Subsystem/Turbine Dynamics + Controller/Power controller/Kω2 controller/Pitch controller/   ==
  rpm : Inport
  Multiply : Gain  Gain=2 * pi
  Multiply1 : Gain  Gain=1 / 60
  rad/s : Outport
  wires:
  Multiply1/1 -> rad/s/1
  rpm/1 -> Multiply/1
  Multiply/1 -> Multiply1/1

== system wturbines/For Each Subsystem/Turbine Dynamics + Controller/Power controller/Kω2 controller/Pitch controller/rad2deg ==
  deg : Inport
  Degrees to Radians : simulink_extras/Transformations/Degrees to Radians
  rad : Outport
  wires:
  Degrees to Radians/1 -> rad/1
  deg/1 -> Degrees to Radians/1

== system wturbines/For Each Subsystem/Turbine Dynamics + Controller1/Control logic/Power controller/Gain-scheduled H∞ control /  ==
  rpm : Inport
  Multiply : Gain  Gain=2 * pi
  Multiply1 : Gain  Gain=1 / 60
  rad/s : Outport
  wires:
  Multiply/1 -> Multiply1/1
  rpm/1 -> Multiply/1
  Multiply1/1 -> rad/s/1

== system wturbines/For Each Subsystem/Turbine Dynamics + Controller1/Control logic/Power controller/Gain-scheduled H∞ control /   ==
  rpm : Inport
  Multiply : Gain  Gain=2 * pi
  Multiply1 : Gain  Gain=1 / 60
  rad/s : Outport
  wires:
  Multiply/1 -> Multiply1/1
  rpm/1 -> Multiply/1
  Multiply1/1 -> rad/s/1

== system wturbines/For Each Subsystem/Turbine Dynamics + Controller1/Control logic/Power controller/Gain-scheduled H∞ control /Pitch controller ==
  e_ω,r(t) : Inport
  β(t) : Inport  Port=2
  Bus Creator : BusCreator  Inputs=2
  Gain : Gain  Gain=K_p_pitch_gs
  Gain scheduler : slctrl_autotuning/PID Gain Scheduler  ControllerType=PI  BPsInGainArray=off  GainArrayBreakpoints=[0 30]  UseExternalBreakpoints=off  GainSourceMethod=Input to block  StoreGainsPParamName=PGain  StoreGainsIParamName=IGain  StoreGainsDParamName=DGain  StoreGainsNParamName=NGain  BlockDataType=Double  PGainLookUpMeth=Interpolation-Use End Values  IGainLookUpMeth=Interpolation-Use End Values  DGainLookUpMeth=Interpolation-Use End Values  NGainLookUpMeth=Interpolation-Use End Values  DoSatur=off  BreakpointSourceLookupVariant=InternalBPs  GainSourceVariant=External  BreakpointSourceVariant=InternalBPs  PGainVariant=Enabled  IGainVariant=Enabled  DGainVariant=Disabled  NGainVariant=Disabled
      settings: LibrarySourceBlock=slctrlblks/Autotuning/PID Gain Scheduler
  Gain1 : Gain  Gain=K_i_pitch_gs
  Gains : Constant  Value=[1 3]
  PI Controller : slpidlib/PID Controller  Controller=PI  Form=Parallel  TimeDomain=Continuous-time  UseExternalTs=off  SampleTime=-1  IntegratorMethod=Forward Euler  FilterMethod=Forward Euler  ControllerParametersSource=external  P=1  I=1  UseKiTs=off  D=0  UseExternalDerivativeSource=off  N=100  UseFilter=on  TunerSelectOption=Transfer Function Based (PID Tuner App)  InitialConditionSource=internal  InitialConditionForIntegrator=0  InitialConditionForFilter=0  DifferentiatorICPrevScaledInput=0  ExternalReset=none  TrackingMode=off  Kt=1  LimitOutput=off  SatLimitsSource=internal  UpperSaturationLimit=inf  LowerSaturationLimit=-inf  LinearizeAsGain=on  AntiWindupMode=none  Kb=1  LimitIntegrator=off  UpperIntegratorSaturationLimit=inf  LowerIntegratorSaturationLimit=-inf  POutMin=[]  POutMax=[]  IOutMin=[]  IOutMax=[]  DOutMin=[]  DOutMax=[]  NOutMin=[]  NOutMax=[]  SumOutMin=[]  SumOutMax=[]  SaturationOutMin=[]  SaturationOutMax=[]  PParamMin=[]  PParamMax=[]  IParamMin=[]  IParamMax=[]  DParamMin=[]  DParamMax=[]  NParamMin=[]  NParamMax=[]  KbParamMin=[]  KbParamMax=[]  KtParamMin=[]  KtParamMax=[]  KbOutMin=[]  KbOutMax=[]  KtOutMin=[]  KtOutMax=[]  IntegratorOutMin=[]  IntegratorOutMax=[]  FilterOutMin=[]  FilterOutMax=[]  SumI1OutMin=[]  SumI1OutMax=[]  SumI2OutMin=[]  SumI2OutMax=[]  SumI3OutMin=[]  SumI3OutMax=[]  SumI4OutMin=[]  SumI4OutMax=[]  SumDOutMin=[]  SumDOutMax=[]  DifferentiatorOutMin=[]  DifferentiatorOutMax=[]  FilterDiffOutCoefMin=[]  FilterDiffOutCoefMax=[]  ReciprocalOutMin=[]  ReciprocalOutMax=[]  SumDenOutMin=[]  SumDenOutMax=[]  SumNumOutMin=[]  SumNumOutMax=[]  DivideOutMin=[]  DivideOutMax=[]  UdiffTsProdOutMin=[]  UdiffTsProdOutMax=[]  NTsProdOutMin=[]  NTsProdOutMax=[]  UintegralTsProdOutMin=[]  UintegralTsProdOutMax=[]  UngainTsProdOutMin=[]  UngainTsProdOutMax=[]  ClampingZeroOutDataTypeStr=Inherit: Inherit via back propagation  ClampingZeroOutMin=[]  ClampingZeroOutMax=[]  FilterDenConstantOutDataTypeStr=Inherit: Inherit via back propagation  FilterDenConstantOutMin=[]  FilterDenConstantOutMax=[]  PCopyOutDataTypeStr=Inherit: Inherit via back propagation  PCopyOutMin=[]  PCopyOutMax=[]  NCopyOutDataTypeStr=Inherit: Inherit via back propagation  NCopyOutMin=[]  NCopyOutMax=[]  IntegratorContinuousStateAttributes=''  IntegratorStateMustResolveToSignalObject=off  IntegratorRTWStateStorageClass=Auto  FilterContinuousStateAttributes=''  FilterStateMustResolveToSignalObject=off  FilterRTWStateStorageClass=Auto  ParallelPVariant=ExternalParameters  IdealPVariant=Disabled  IVariant=ExternalParameters  DVariant=Disabled  IntegratorVariant=Continuous  SatVariant=Disabled  AWVariant=Passthrough  PCopyVariant=Disabled  TRVariant=Disabled  FdbkBlocksVariant=Forward  IdealPFdbkVariant=Disabled  SatFdbkVariant=Disabled  DerivativeFilterVariant=Disabled  NVariant=Disabled  NCopyVariant=Disabled_SignalSpec  FilterICVariant=Disabled  IntegratorICVariant=InternalICs  ExternalResetVariant=Disabled  TRSumVariant=Passthrough  SumFdbkVariant=Disabled  SumVariant=Sum_PI  TsampFilterVariant=InternalTs  TsampNgainVariant=Passthrough  TsampIntegralVariant=Disabled_SignalSpec  ExternalSaturationOutDataTypeStr=Inherit: Same as second input  DerivativeSourceVariant=Disabled  PreIntVariant=InternalPreInt
  Signal Copy : SignalConversion  OverrideOpt=off
  rad2deg : Subsystem
  β_ref(t) : Outport
  wires:
  e_ω,r(t)/1 -> PI Controller/1
  PI Controller/1 -> β_ref(t)/1
  Gain scheduler/1 -> Gain/1
  Gain scheduler/2 -> Gain1/1
  Gain/1 -> PI Controller/2
  Gain1/1 -> PI Controller/3
  Bus Creator/1 -> Gain scheduler/2
  Gains/1 -> Signal Copy/1, Bus Creator/1  "P"
  rad2deg/1(deg) -> Gain scheduler/1  "β(t)"
  β(t)/1 -> rad2deg/1(rad)
  Signal Copy/1 -> Bus Creator/2  "I"

== system wturbines/For Each Subsystem/Turbine Dynamics + Controller1/Control logic/Power controller/Gain-scheduled H∞ control /Torque controller ==
  note: Temporary workaround
  e_ω,r(t) : Inport
  "H∞ controller " : StateSpace  A=A_k  B=B_k  C=C_k  D=D_k  InitialCondition=0
  PI controller : slpidlib/PID Controller  Controller=PI  Form=Parallel  TimeDomain=Continuous-time  UseExternalTs=off  SampleTime=-1  IntegratorMethod=Forward Euler  FilterMethod=Forward Euler  ControllerParametersSource=internal  P=A_k  I=B_k  UseKiTs=off  D=0  UseExternalDerivativeSource=off  N=100  UseFilter=on  TunerSelectOption=Transfer Function Based (PID Tuner App)  InitialConditionSource=internal  InitialConditionForIntegrator=0  InitialConditionForFilter=0  DifferentiatorICPrevScaledInput=0  ExternalReset=none  TrackingMode=off  Kt=1  LimitOutput=off  SatLimitsSource=internal  UpperSaturationLimit=inf  LowerSaturationLimit=-inf  LinearizeAsGain=on  AntiWindupMode=none  Kb=1  LimitIntegrator=off  UpperIntegratorSaturationLimit=inf  LowerIntegratorSaturationLimit=-inf  POutMin=[]  POutMax=[]  IOutMin=[]  IOutMax=[]  DOutMin=[]  DOutMax=[]  NOutMin=[]  NOutMax=[]  SumOutMin=[]  SumOutMax=[]  SaturationOutMin=[]  SaturationOutMax=[]  PParamMin=[]  PParamMax=[]  IParamMin=[]  IParamMax=[]  DParamMin=[]  DParamMax=[]  NParamMin=[]  NParamMax=[]  KbParamMin=[]  KbParamMax=[]  KtParamMin=[]  KtParamMax=[]  KbOutMin=[]  KbOutMax=[]  KtOutMin=[]  KtOutMax=[]  IntegratorOutMin=[]  IntegratorOutMax=[]  FilterOutMin=[]  FilterOutMax=[]  SumI1OutMin=[]  SumI1OutMax=[]  SumI2OutMin=[]  SumI2OutMax=[]  SumI3OutMin=[]  SumI3OutMax=[]  SumI4OutMin=[]  SumI4OutMax=[]  SumDOutMin=[]  SumDOutMax=[]  DifferentiatorOutMin=[]  DifferentiatorOutMax=[]  FilterDiffOutCoefMin=[]  FilterDiffOutCoefMax=[]  ReciprocalOutMin=[]  ReciprocalOutMax=[]  SumDenOutMin=[]  SumDenOutMax=[]  SumNumOutMin=[]  SumNumOutMax=[]  DivideOutMin=[]  DivideOutMax=[]  UdiffTsProdOutMin=[]  UdiffTsProdOutMax=[]  NTsProdOutMin=[]  NTsProdOutMax=[]  UintegralTsProdOutMin=[]  UintegralTsProdOutMax=[]  UngainTsProdOutMin=[]  UngainTsProdOutMax=[]  ClampingZeroOutDataTypeStr=Inherit: Inherit via back propagation  ClampingZeroOutMin=[]  ClampingZeroOutMax=[]  FilterDenConstantOutDataTypeStr=Inherit: Inherit via back propagation  FilterDenConstantOutMin=[]  FilterDenConstantOutMax=[]  PCopyOutDataTypeStr=Inherit: Inherit via back propagation  PCopyOutMin=[]  PCopyOutMax=[]  NCopyOutDataTypeStr=Inherit: Inherit via back propagation  NCopyOutMin=[]  NCopyOutMax=[]  IntegratorContinuousStateAttributes=''  IntegratorStateMustResolveToSignalObject=off  IntegratorRTWStateStorageClass=Auto  FilterContinuousStateAttributes=''  FilterStateMustResolveToSignalObject=off  FilterRTWStateStorageClass=Auto  ParallelPVariant=InternalParameters  IdealPVariant=Disabled  IVariant=InternalParameters  DVariant=Disabled  IntegratorVariant=Continuous  SatVariant=Disabled  AWVariant=Passthrough  PCopyVariant=Disabled  TRVariant=Disabled  FdbkBlocksVariant=Forward  IdealPFdbkVariant=Disabled  SatFdbkVariant=Disabled  DerivativeFilterVariant=Disabled  NVariant=Disabled  NCopyVariant=Disabled_SignalSpec  FilterICVariant=Disabled  IntegratorICVariant=InternalICs  ExternalResetVariant=Disabled  TRSumVariant=Passthrough  SumFdbkVariant=Disabled  SumVariant=Sum_PI  TsampFilterVariant=InternalTs  TsampNgainVariant=Passthrough  TsampIntegralVariant=Disabled_SignalSpec  ExternalSaturationOutDataTypeStr=Inherit: Same as second input  DerivativeSourceVariant=Disabled  PreIntVariant=InternalPreInt
  T_g(t) : Outport
  wires:
  e_ω,r(t)/1 -> PI controller/1
  PI controller/1 -> T_g(t)/1
  "H∞ controller "/1 -> ?

== system wturbines/For Each Subsystem/Turbine Dynamics + Controller1/Control logic/Power controller/Kω2 controller/Pitch controller ==
  ws(t) : Inport
  ω(t) : Inport  Port=2
  "  " : Subsystem
  Constant : Constant  Value=rated_rotor_speed
  Constant1 : Constant  Value=alpha_pitch_exp
  Constant2 : Constant  Value=0
  Exp : Math
  Gain : Gain
  IsNaN1 : RelationalOperator  Operator=isNaN  OutDataTypeStr=boolean  RndMeth=Simplest  InputSameDT=off
  NOT : Logic  Operator=NOT  IconShape=distinctive  AllPortsSameDT=off  OutDataTypeStr=boolean
  Product : Product
  Product1 : Product
  Sum : Sum  Inputs=|+-
  Switch : Switch  Criteria=u2 ~= 0  SaturateOnIntegerOverflow=off  InputSameDT=off
  rad2deg : Subsystem
  β(ws) : Lookup_n-D  NumberOfTableDimensions=1  BreakpointsForDimension1=u_all  Table=pitch_all  ExtrapMethod=Clip  UseLastTableValue=on  InternalRulePriority=Speed  RndMeth=Simplest
  β(t) : Outport
  wires:
  β(ws)/1 -> rad2deg/1(deg)
  ws(t)/1 -> β(ws)/1
  ω(t)/1 -> Sum/1
  Constant/1 -> "  "/1(rpm)
  Exp/1 -> Product/2
  Sum/1 -> Product1/1
  Product1/1 -> Exp/1
  Constant1/1 -> IsNaN1/1, Product1/2
  rad2deg/1(rad) -> Gain/1  "β(t)"
  "  "/1(rad/s) -> Sum/2  "ω_rated"
  IsNaN1/1 -> NOT/1
  Constant2/1 -> Switch/3
  Product/1 -> Switch/1
  NOT/1 -> Switch/2  "is_not_nan"
  Switch/1 -> β(t)/1
  Gain/1 -> Product/1

== system wturbines/For Each Subsystem/Turbine Dynamics + Controller1/Control logic/Power controller/Kω2 controller/Torque controller ==
  ω(t) : Inport
  ws : Inport  Port=2
  Constant : Constant  Value=K_omega_sq
  Constant1 : Constant  Value=rated_power / (rated_rotor_speed_rads * gearbox_ratio)
  Product : Product
  Relay : Relay  OnSwitchValue=rated_wind_speed  OffSwitchValue=rated_wind_speed - 1
  Square : Math  Operator=square
  Switch : Switch  Criteria=u2 > Threshold  SaturateOnIntegerOverflow=off  InputSameDT=off
  T_g(t) : Outport
  wires:
  ω(t)/1 -> Square/1
  Square/1 -> Product/1
  Product/1 -> T_g(t)/1, Switch/3
  Constant/1 -> Product/2
  ws/1 -> Relay/1
  Relay/1 -> Switch/2
  Constant1/1 -> Switch/1

== system wturbines/For Each Subsystem/Turbine Dynamics + Controller1/Control logic/Power controller/Lio downregulation/   ==
  rpm : Inport
  Multiply : Gain  Gain=2 * pi
  Multiply1 : Gain  Gain=1 / 60
  rad/s : Outport
  wires:
  Multiply/1 -> Multiply1/1
  rpm/1 -> Multiply/1
  Multiply1/1 -> rad/s/1
